simulink model "s_c_nbe_m32k"  (R2018a)
settings: Solver=VariableStepDiscrete  StartTime=0.0  StopTime=1000  RelTol=1e-3
undefined symbols (not defined in the file): fft_stages, n_taps, output_bits, pfb_coeff_gen_calc, xengbits
libraries: xbsIndex_r4 x23714, casper_library_misc x17, xps_library x4, casper_library_scopes x4, xbsReplacements_r4 x4
(part 62 of 171)

== system s_c_nbe_m32k/wb_prog_delay/delay_wideband_prog ==
  sync : Inport
  delay : Inport  Port=2
  ld_delay : Inport  Port=3
  data_in0 : Inport  Port=4
  data_in1 : Inport  Port=5
  data_in2 : Inport  Port=6
  data_in3 : Inport  Port=7
  data_in4 : Inport  Port=8
  data_in5 : Inport  Port=9
  data_in6 : Inport  Port=10
  data_in7 : Inport  Port=11
  en : Inport  Port=12
  AddSub{1..7} (7 alike) : xbsIndex_r4/AddSub  mode=Addition  use_carryin=off  use_carryout=off  en=off  latency=0  precision=Full  arith_type=Unsigned  n_bits=1  bin_pt=0  quantization=Truncate  overflow=Wrap  use_behavioral_HDL=off  hw_selection=Fabric  pipelined=off  dbl_ovrd=off  block_type=addsub
  Constant1 : xbsIndex_r4/Constant  const=6  gui_display_data_type=Fixed-point  arith_type=Unsigned  n_bits=3  bin_pt=0  preci_type=Single  exp_width=8  frac_width=24  explicit_period=on  period=1  equ=P=C  opselect=C  inp2=PCIN>>17  opr=+  inp1=P  carry=CIN  dbl_ovrd=off  block_type=constant
  Constant2 : xbsIndex_r4/Constant  const=5  gui_display_data_type=Fixed-point  arith_type=Unsigned  n_bits=3  bin_pt=0  preci_type=Single  exp_width=8  frac_width=24  explicit_period=on  period=1  equ=P=C  opselect=C  inp2=PCIN>>17  opr=+  inp1=P  carry=CIN  dbl_ovrd=off  block_type=constant
  Constant3 : xbsIndex_r4/Constant  const=4  gui_display_data_type=Fixed-point  arith_type=Unsigned  n_bits=3  bin_pt=0  preci_type=Single  exp_width=8  frac_width=24  explicit_period=on  period=1  equ=P=C  opselect=C  inp2=PCIN>>17  opr=+  inp1=P  carry=CIN  dbl_ovrd=off  block_type=constant
  Constant4 : xbsIndex_r4/Constant  const=3  gui_display_data_type=Fixed-point  arith_type=Unsigned  n_bits=3  bin_pt=0  preci_type=Single  exp_width=8  frac_width=24  explicit_period=on  period=1  equ=P=C  opselect=C  inp2=PCIN>>17  opr=+  inp1=P  carry=CIN  dbl_ovrd=off  block_type=constant
  Constant5 : xbsIndex_r4/Constant  const=2  gui_display_data_type=Fixed-point  arith_type=Unsigned  n_bits=3  bin_pt=0  preci_type=Single  exp_width=8  frac_width=24  explicit_period=on  period=1  equ=P=C  opselect=C  inp2=PCIN>>17  opr=+  inp1=P  carry=CIN  dbl_ovrd=off  block_type=constant
  Constant6 : xbsIndex_r4/Constant  const=1  gui_display_data_type=Fixed-point  arith_type=Unsigned  n_bits=3  bin_pt=0  preci_type=Single  exp_width=8  frac_width=24  explicit_period=on  period=1  equ=P=C  opselect=C  inp2=PCIN>>17  opr=+  inp1=P  carry=CIN  dbl_ovrd=off  block_type=constant
  Constant7 : xbsIndex_r4/Constant  const=0  gui_display_data_type=Fixed-point  arith_type=Unsigned  n_bits=3  bin_pt=0  preci_type=Single  exp_width=8  frac_width=24  explicit_period=on  period=1  equ=P=C  opselect=C  inp2=PCIN>>17  opr=+  inp1=P  carry=CIN  dbl_ovrd=off  block_type=constant
  Convert{1..7} (7 alike) : xbsIndex_r4/Convert  gui_display_data_type=Fixed-point  arith_type=Unsigned  n_bits=1  bin_pt=0  float_type=Single  exp_bits=8  fraction_bits=24  quantization=Truncate  overflow=Wrap  en=off  latency=0  pipeline=off  dbl_ovrd=off  block_type=convert
  Relational{1..7} (7 alike) : xbsIndex_r4/Relational  mode=a>b  op_type=Bool  en=off  latency=0  dbl_ovrd=off  block_type=relational
  barrel_switcher : Subsystem  mask(barrel_switcher){n_inputs=3, async=on}
      mask prompts: n_inputs "Number of Inputs: (2^?)"; async "Asynchronous operation"
      mask help:
      | Shifts input to right by amount specified on sel,
      | wrapping around into higher order bits.
      mask init:
      | barrel_switcher_init(gcb,...
      |     'n_inputs', n_inputs, ...
      |     'async', async);
      mask Help: eval('xlWeb(''http://casper.berkeley.edu/wiki/Barrel_switcher'')')
  bram_rd_addrs : xbsIndex_r4/Slice  nbits=1  boolean_output=off  mode=Lower Bit Location + Width  bit1=0  base1=MSB of Input  bit0=3  base0=LSB of Input  dbl_ovrd=off  block_type=slice
  delay_dp0 : Subsystem  mask(delay_bram_prog_dp){ram_bits=2, bram_latency=3, async=on}
      mask prompts: ram_bits "Max delay (2^?)"; bram_latency "BRAM latency"; async "asynchronous operation"
      mask init:
      | %delay_bram_prog_dp_init(gcb, ...
      | %    'ram_bits', ram_bits, ...
      | %    'bram_latency', bram_latency, ...
      | %    'async', async);
  delay_dp1 : Subsystem  mask(delay_bram_prog_dp){ram_bits=2, bram_latency=3, async=on}
      mask prompts: ram_bits "Max delay (2^?)"; bram_latency "BRAM latency"; async "asynchronous operation"
      mask init:
      | %delay_bram_prog_dp_init(gcb, ...
      | %    'ram_bits', ram_bits, ...
      | %    'bram_latency', bram_latency, ...
      | %    'async', async);
  delay_dp2 : Subsystem  mask(delay_bram_prog_dp){ram_bits=2, bram_latency=3, async=on}
      mask prompts: ram_bits "Max delay (2^?)"; bram_latency "BRAM latency"; async "asynchronous operation"
      mask init:
      | %delay_bram_prog_dp_init(gcb, ...
      | %    'ram_bits', ram_bits, ...
      | %    'bram_latency', bram_latency, ...
      | %    'async', async);
  delay_dp3 : Subsystem  mask(delay_bram_prog_dp){ram_bits=2, bram_latency=3, async=on}
      mask prompts: ram_bits "Max delay (2^?)"; bram_latency "BRAM latency"; async "asynchronous operation"
      mask init:
      | %delay_bram_prog_dp_init(gcb, ...
      | %    'ram_bits', ram_bits, ...
      | %    'bram_latency', bram_latency, ...
      | %    'async', async);
  delay_dp4 : Subsystem  mask(delay_bram_prog_dp){ram_bits=2, bram_latency=3, async=on}
      mask prompts: ram_bits "Max delay (2^?)"; bram_latency "BRAM latency"; async "asynchronous operation"
      mask init:
      | %delay_bram_prog_dp_init(gcb, ...
      | %    'ram_bits', ram_bits, ...
      | %    'bram_latency', bram_latency, ...
      | %    'async', async);
  delay_dp5 : Subsystem  mask(delay_bram_prog_dp){ram_bits=2, bram_latency=3, async=on}
      mask prompts: ram_bits "Max delay (2^?)"; bram_latency "BRAM latency"; async "asynchronous operation"
      mask init:
      | %delay_bram_prog_dp_init(gcb, ...
      | %    'ram_bits', ram_bits, ...
      | %    'bram_latency', bram_latency, ...
      | %    'async', async);
  delay_dp6 : Subsystem  mask(delay_bram_prog_dp){ram_bits=2, bram_latency=3, async=on}
      mask prompts: ram_bits "Max delay (2^?)"; bram_latency "BRAM latency"; async "asynchronous operation"
      mask init:
      | %delay_bram_prog_dp_init(gcb, ...
      | %    'ram_bits', ram_bits, ...
      | %    'bram_latency', bram_latency, ...
      | %    'async', async);
  delay_dp7 : Subsystem  mask(delay_bram_prog_dp){ram_bits=2, bram_latency=3, async=on}
      mask prompts: ram_bits "Max delay (2^?)"; bram_latency "BRAM latency"; async "asynchronous operation"
      mask init:
      | %delay_bram_prog_dp_init(gcb, ...
      | %    'ram_bits', ram_bits, ...
      | %    'bram_latency', bram_latency, ...
      | %    'async', async);
  delay_reg : xbsIndex_r4/Register  init=0  rst=off  en=on  dbl_ovrd=off  block_type=register
  delay_sel : xbsIndex_r4/Delay  rst=off  infoeditControl=Selection of Reset will increase slice count due to use of real FFs and instead of SRLs  en=off  latency=4  reg_retiming=on  dbl_ovrd=off  block_type=delay
  en_delay0 : xbsIndex_r4/Delay  rst=off  infoeditControl=Selection of Reset will increase slice count due to use of real FFs and instead of SRLs  en=off  latency=0  reg_retiming=on  dbl_ovrd=off  block_type=delay
  en_delay1 : xbsIndex_r4/Delay  rst=off  infoeditControl=Selection of Reset will increase slice count due to use of real FFs and instead of SRLs  en=off  latency=4  reg_retiming=on  dbl_ovrd=off  block_type=delay
  shift_sel : xbsIndex_r4/Slice  nbits=3  boolean_output=off  mode=Lower Bit Location + Width  bit1=0  base1=MSB of Input  bit0=0  base0=LSB of Input  dbl_ovrd=off  block_type=slice
  sync_delay : xbsIndex_r4/Delay  rst=off  infoeditControl=Selection of Reset will increase slice count due to use of real FFs and instead of SRLs  en=off  latency=4  reg_retiming=on  dbl_ovrd=off  block_type=delay
  sync_out : Outport
  data_out0 : Outport  Port=2
  data_out1 : Outport  Port=3
  data_out2 : Outport  Port=4
  data_out3 : Outport  Port=5
  data_out4 : Outport  Port=6
  data_out5 : Outport  Port=7
  data_out6 : Outport  Port=8
  data_out7 : Outport  Port=9
  dvalid : Outport  Port=10
  wires:
  en/1 -> en_delay0/1
  en_delay0/1 -> en_delay1/1, delay_dp0/3(en), delay_dp1/3(en), delay_dp2/3(en), delay_dp3/3(en), delay_dp4/3(en), delay_dp5/3(en), delay_dp6/3(en), delay_dp7/3(en)  "dp_en"
  sync/1 -> sync_delay/1
  delay/1 -> delay_reg/1
  ld_delay/1 -> delay_reg/2
  delay_reg/1 -> bram_rd_addrs/1, shift_sel/1
  sync_delay/1 -> barrel_switcher/2(sync_in)
  barrel_switcher/1(sync_out) -> sync_out/1
  en_delay1/1 -> barrel_switcher/11(en)
  barrel_switcher/10(dvalid) -> dvalid/1
  shift_sel/1 -> delay_sel/1, Relational1/1, Relational2/1, Relational3/1, Relational4/1, Relational5/1, Relational6/1, Relational7/1
  delay_sel/1 -> barrel_switcher/1(sel)
  barrel_switcher/9(Out8) -> data_out0/1
  barrel_switcher/8(Out7) -> data_out1/1
  barrel_switcher/7(Out6) -> data_out2/1
  barrel_switcher/6(Out5) -> data_out3/1
  barrel_switcher/5(Out4) -> data_out4/1
  barrel_switcher/4(Out3) -> data_out5/1
  barrel_switcher/3(Out2) -> data_out6/1
  barrel_switcher/2(Out1) -> data_out7/1
  data_in0/1 -> delay_dp0/1(din)  "dp_val0"
  delay_dp0/1(dout) -> barrel_switcher/10(In8)
  bram_rd_addrs/1 -> delay_dp0/2(delay), AddSub1/1, AddSub2/1, AddSub3/1, AddSub4/1, AddSub5/1, AddSub6/1, AddSub7/1  "dp0"
  data_in1/1 -> delay_dp1/1(din)  "dp_val1"
  delay_dp1/1(dout) -> barrel_switcher/9(In7)
  Constant1/1 -> Relational1/2
  Relational1/1 -> Convert1/1
  Convert1/1 -> AddSub1/2
  AddSub1/1 -> delay_dp1/2(delay)  "dp1"
  data_in2/1 -> delay_dp2/1(din)  "dp_val2"
  delay_dp2/1(dout) -> barrel_switcher/8(In6)
  Constant2/1 -> Relational2/2
  Relational2/1 -> Convert2/1
  Convert2/1 -> AddSub2/2
  AddSub2/1 -> delay_dp2/2(delay)  "dp2"
  data_in3/1 -> delay_dp3/1(din)  "dp_val3"
  delay_dp3/1(dout) -> barrel_switcher/7(In5)
  Constant3/1 -> Relational3/2
  Relational3/1 -> Convert3/1
  Convert3/1 -> AddSub3/2
  AddSub3/1 -> delay_dp3/2(delay)  "dp3"
  data_in4/1 -> delay_dp4/1(din)  "dp_val4"
  delay_dp4/1(dout) -> barrel_switcher/6(In4)
  Constant4/1 -> Relational4/2
  Relational4/1 -> Convert4/1
  Convert4/1 -> AddSub4/2
  AddSub4/1 -> delay_dp4/2(delay)  "dp4"
  data_in5/1 -> delay_dp5/1(din)  "dp_val5"
  delay_dp5/1(dout) -> barrel_switcher/5(In3)
  Constant5/1 -> Relational5/2
  Relational5/1 -> Convert5/1
  Convert5/1 -> AddSub5/2
  AddSub5/1 -> delay_dp5/2(delay)  "dp5"
  data_in6/1 -> delay_dp6/1(din)  "dp_val6"
  delay_dp6/1(dout) -> barrel_switcher/4(In2)
  Constant6/1 -> Relational6/2
  Relational6/1 -> Convert6/1
  Convert6/1 -> AddSub6/2
  AddSub6/1 -> delay_dp6/2(delay)  "dp6"
  data_in7/1 -> delay_dp7/1(din)  "dp_val7"
  delay_dp7/1(dout) -> barrel_switcher/3(In1)
  Constant7/1 -> Relational7/2
  Relational7/1 -> Convert7/1
  Convert7/1 -> AddSub7/2
  AddSub7/1 -> delay_dp7/2(delay)  "dp7"

== system s_c_nbe_m32k/wb_prog_delay1/bus_expand ==
  bus_in : Inport
  reinterpret{1..8} (8 alike) : xbsIndex_r4/Reinterpret  force_arith_type=on  arith_type=Unsigned  force_bin_pt=on  bin_pt=0  block_type=reinterpret
  slice1 : xbsIndex_r4/Slice  nbits=10  boolean_output=off  mode=Upper Bit Location + Width  bit1=-70  base1=MSB of Input  bit0=0  base0=LSB of Input  dbl_ovrd=off  block_type=slice
  slice2 : xbsIndex_r4/Slice  nbits=10  boolean_output=off  mode=Upper Bit Location + Width  bit1=-60  base1=MSB of Input  bit0=0  base0=LSB of Input  dbl_ovrd=off  block_type=slice
  slice3 : xbsIndex_r4/Slice  nbits=10  boolean_output=off  mode=Upper Bit Location + Width  bit1=-50  base1=MSB of Input  bit0=0  base0=LSB of Input  dbl_ovrd=off  block_type=slice
  slice4 : xbsIndex_r4/Slice  nbits=10  boolean_output=off  mode=Upper Bit Location + Width  bit1=-40  base1=MSB of Input  bit0=0  base0=LSB of Input  dbl_ovrd=off  block_type=slice
  slice5 : xbsIndex_r4/Slice  nbits=10  boolean_output=off  mode=Upper Bit Location + Width  bit1=-30  base1=MSB of Input  bit0=0  base0=LSB of Input  dbl_ovrd=off  block_type=slice
  slice6 : xbsIndex_r4/Slice  nbits=10  boolean_output=off  mode=Upper Bit Location + Width  bit1=-20  base1=MSB of Input  bit0=0  base0=LSB of Input  dbl_ovrd=off  block_type=slice
  slice7 : xbsIndex_r4/Slice  nbits=10  boolean_output=off  mode=Upper Bit Location + Width  bit1=-10  base1=MSB of Input  bit0=0  base0=LSB of Input  dbl_ovrd=off  block_type=slice
  slice8 : xbsIndex_r4/Slice  nbits=10  boolean_output=off  mode=Upper Bit Location + Width  bit1=0  base1=MSB of Input  bit0=0  base0=LSB of Input  dbl_ovrd=off  block_type=slice
  msb_out8 : Outport
  out7 : Outport  Port=2
  out6 : Outport  Port=3
  out5 : Outport  Port=4
  out4 : Outport  Port=5
  out3 : Outport  Port=6
  out2 : Outport  Port=7
  lsb_out1 : Outport  Port=8
  wires:
  bus_in/1 -> slice8/1, slice7/1, slice6/1, slice5/1, slice4/1, slice3/1, slice2/1, slice1/1
  slice8/1 -> reinterpret8/1
  reinterpret8/1 -> msb_out8/1
  slice7/1 -> reinterpret7/1
  reinterpret7/1 -> out7/1
  slice6/1 -> reinterpret6/1
  reinterpret6/1 -> out6/1
  slice5/1 -> reinterpret5/1
  reinterpret5/1 -> out5/1
  slice4/1 -> reinterpret4/1
  reinterpret4/1 -> out4/1
  slice3/1 -> reinterpret3/1
  reinterpret3/1 -> out3/1
  slice2/1 -> reinterpret2/1
  reinterpret2/1 -> out2/1
  slice1/1 -> reinterpret1/1
  reinterpret1/1 -> lsb_out1/1

== system s_c_nbe_m32k/wb_prog_delay1/bus_expand1 ==
  bus_in : Inport
  reinterpret1 : xbsIndex_r4/Reinterpret  force_arith_type=on  arith_type="Signed  (2's comp)"  force_bin_pt=on  bin_pt=15  block_type=reinterpret
  reinterpret2 : xbsIndex_r4/Reinterpret  force_arith_type=on  arith_type="Signed  (2's comp)"  force_bin_pt=on  bin_pt=15  block_type=reinterpret
  reinterpret3 : xbsIndex_r4/Reinterpret  force_arith_type=on  arith_type="Signed  (2's comp)"  force_bin_pt=on  bin_pt=32  block_type=reinterpret
  reinterpret4 : xbsIndex_r4/Reinterpret  force_arith_type=on  arith_type="Signed  (2's comp)"  force_bin_pt=on  bin_pt=32  block_type=reinterpret
  slice1 : xbsIndex_r4/Slice  nbits=16  boolean_output=off  mode=Upper Bit Location + Width  bit1=-144  base1=MSB of Input  bit0=0  base0=LSB of Input  dbl_ovrd=off  block_type=slice
  slice2 : xbsIndex_r4/Slice  nbits=16  boolean_output=off  mode=Upper Bit Location + Width  bit1=-128  base1=MSB of Input  bit0=0  base0=LSB of Input  dbl_ovrd=off  block_type=slice
  slice3 : xbsIndex_r4/Slice  nbits=64  boolean_output=off  mode=Upper Bit Location + Width  bit1=-64  base1=MSB of Input  bit0=0  base0=LSB of Input  dbl_ovrd=off  block_type=slice
  slice4 : xbsIndex_r4/Slice  nbits=64  boolean_output=off  mode=Upper Bit Location + Width  bit1=0  base1=MSB of Input  bit0=0  base0=LSB of Input  dbl_ovrd=off  block_type=slice
  msb_out4 : Outport
  out3 : Outport  Port=2
  out2 : Outport  Port=3
  lsb_out1 : Outport  Port=4
  wires:
  reinterpret1/1 -> lsb_out1/1
  slice1/1 -> reinterpret1/1
  reinterpret2/1 -> out2/1
  slice2/1 -> reinterpret2/1
  reinterpret3/1 -> out3/1
  slice3/1 -> reinterpret3/1
  reinterpret4/1 -> msb_out4/1
  slice4/1 -> reinterpret4/1
  bus_in/1 -> slice1/1, slice2/1, slice3/1, slice4/1

== system s_c_nbe_m32k/wb_prog_delay1/delay_gen ==
  sync_in : Inport
  din : Inport  Port=2
  en : Inport  Port=3
  delay : Inport  Port=4
  d/dt_delay : Inport  Port=5
  phase : Inport  Port=6
  d/dt_phase : Inport  Port=7
  ld : Inport  Port=8
  Constant : xbsIndex_r4/Constant  const=2^(n_bits_fft_words-1)  gui_display_data_type=Fixed-point  arith_type=Unsigned  n_bits=n_bits_fft_words  bin_pt=0  preci_type=Single  exp_width=8  frac_width=24  explicit_period=on  period=1  equ=P=C  opselect=C  inp2=PCIN>>17  opr=+  inp1=P  carry=CIN  dbl_ovrd=off  block_type=constant
  Constant53 : xbsIndex_r4/Constant  const=0  gui_display_data_type=Boolean  arith_type=Boolean  n_bits=1  bin_pt=0  preci_type=Single  exp_width=8  frac_width=24  explicit_period=on  period=1  equ=P=C  opselect=C  inp2=PCIN>>17  opr=+  inp1=P  carry=CIN  dbl_ovrd=off  block_type=constant
      settings: block_version=11.4
  Delay{,1..17} (18 alike) : xbsIndex_r4/Delay  rst=off  infoeditControl=Selection of Reset will increase slice count due to use of real FFs and instead of SRLs  en=off  latency=1  reg_retiming=on  dbl_ovrd=off  block_type=delay
  Logical : xbsIndex_r4/Logical  logical_function=AND  inputs=2  en=off  latency=1  precision=Full  arith_type=Unsigned  n_bits=16  bin_pt=0  align_bp=on  dbl_ovrd=off  block_type=logical
  delay_gen : Subsystem  mask{fft_len=n_bits_fft, add_latency=1, data_bits=n_bits_data * 2^n_bits_streams, n_bits_index=n_bits_fft_words, lookup_bits=11, cd_bits=n_bits_cd, delay_bits=n_bits_cd+32, delay_bin_pt=32, max_delay_rate=23, min_delay_rate=38, phase_bits=16, max_phase_rate=23, min_phase_rate=38}
      mask prompts: fft_len "Effective FFT size (2^?)"; add_latency "Add latency"; data_bits "Data width"; n_bits_index "Index width"; lookup_bits "DDS lookup table resolution (2*pi/2^?)"; cd_bits "Coarse delay range (2^? bits)"; delay_bits "Input delay resolution (bits)"; delay_bin_pt "Input delay binary point"; max_delay_rate "Max delay update rate (1/2^? samples/sample)"; min_delay_rate "Min (non-zero) delay update rate (1/2^? samples/sample)"; phase_bits "Input phase resolution (2*pi/2^? radians)"; max_phase_rate "Max phase update rate (1/2^? radians/sample)"; min_phase_rate "Min (non-zero) phase rate (1/2^? radians/sample)"
  edge_detect : Subsystem  mask(edge_detect){edge=Rising, polarity=Active High, x_in=[0 0.08 0.08 0.16 0.16 0.24 0.24 0.32 0.32 0.4], y_in=[-1 -1  1  1  1  1  1  1  1  1], x_out=[0.6 0.68 0.68 0.76 0.76 0.84 0.84 0.92 0.92 1], y_out=[-1 -1  1  1 -1 -1 -1 -1 -1 -1]}
      mask prompts: edge "Edge Type"; polarity "Output Polarity"; x_in "Input X Positions"; y_in "Input Y Positions"; x_out "Output X Positions"; y_out "Output Y Positions"
      mask help: Output is active for one-cycle after each edge of the specified type (i.e. rising, falling or both).
      mask init: same as s_c_nbe_m32k/edge_detect1
      settings: AttributesFormatString=|
      | rising edges
      | active high
      mask Help: Output is active for one-cycle after each edge of the specified type (i.e. rising, falling, or both).  Latency is zero.
      mask TypeOptions edge: Rising | Falling | Both
      mask TypeOptions polarity: Active High | Active Low
      mask Display:
      | plot(x_in_num,0.5+y_in_num*0.2);
      | plot(x_out_num,0.5+y_out_num*0.2);
  fft_index : xbsIndex_r4/Counter  cnt_type=Free Running  cnt_to=Inf  operation=Up  start_count=2^(n_bits_fft_words-1)  cnt_by_val=1  arith_type=Unsigned  n_bits=n_bits_fft_words  bin_pt=0  load_pin=off  rst=on  en=on  explicit_period=on  period=1  use_behavioral_HDL=on  implementation=Fabric  dbl_ovrd=off  block_type=counter
  first : xbsIndex_r4/Relational  mode=a=b  op_type=Bool  en=off  latency=1  dbl_ovrd=off  block_type=relational
  sync_out : Outport
  dout : Outport  Port=2
  idx_out : Outport  Port=3
  dvalid : Outport  Port=4
  initial_phase : Outport  Port=5
  slope : Outport  Port=6
  coarse_delay : Outport  Port=7
  new_value : Outport  Port=8
  wires:
  edge_detect/1(out) -> delay_gen/2(init)
  Logical/1 -> edge_detect/1(in)
  Delay17/1 -> delay_gen/10(d/dt_delay)
  Delay16/1 -> delay_gen/9(delay)
  Delay15/1 -> delay_gen/8(d/dt_phase)
  Delay14/1 -> delay_gen/7(phase)
  Delay13/1 -> delay_gen/6(load)
  Delay12/1 -> delay_gen/5(den)
  Delay11/1 -> delay_gen/4(idx_in)
  Delay10/1 -> delay_gen/3(din)
  Delay9/1 -> delay_gen/1(sync_in)
  Delay1/1 -> Delay10/1
  Delay8/1 -> Delay17/1
  Delay7/1 -> Delay16/1
  Delay6/1 -> Delay15/1
  Delay5/1 -> Delay14/1
  Delay4/1 -> Delay13/1
  delay_gen/8(load_out) -> new_value/1
  delay_gen/7(phase_out) -> initial_phase/1
  delay_gen/6(slope_out) -> slope/1
  delay_gen/5(cd_o) -> coarse_delay/1
  delay_gen/4(dvalid) -> dvalid/1
  delay_gen/3(idx_out) -> idx_out/1
  d/dt_phase/1 -> Delay6/1
  phase/1 -> Delay5/1
  ld/1 -> Delay4/1
  Delay3/1 -> Delay12/1, Logical/2
  Delay2/1 -> Delay11/1
  Delay/1 -> Delay9/1
  first/1 -> Logical/1
  Constant/1 -> first/1
  delay_gen/2(dout) -> dout/1
  en/1 -> fft_index/2, Delay3/1
  d/dt_delay/1 -> Delay8/1
  delay_gen/1(sync_out) -> sync_out/1
  delay/1 -> Delay7/1
  fft_index/1 -> first/2, Delay2/1
  Constant53/1 -> delay_gen/11(invert_slope)
  sync_in/1 -> fft_index/1, Delay/1
  din/1 -> Delay1/1

== system s_c_nbe_m32k/wb_prog_delay1/delay_wideband_prog ==
  sync : Inport
  delay : Inport  Port=2
  ld_delay : Inport  Port=3
  data_in0 : Inport  Port=4
  data_in1 : Inport  Port=5
  data_in2 : Inport  Port=6
  data_in3 : Inport  Port=7
  data_in4 : Inport  Port=8
  data_in5 : Inport  Port=9
  data_in6 : Inport  Port=10
  data_in7 : Inport  Port=11
  en : Inport  Port=12
  AddSub{1..7} (7 alike) : xbsIndex_r4/AddSub  mode=Addition  use_carryin=off  use_carryout=off  en=off  latency=0  precision=Full  arith_type=Unsigned  n_bits=1  bin_pt=0  quantization=Truncate  overflow=Wrap  use_behavioral_HDL=off  hw_selection=Fabric  pipelined=off  dbl_ovrd=off  block_type=addsub
  Constant1 : xbsIndex_r4/Constant  const=6  gui_display_data_type=Fixed-point  arith_type=Unsigned  n_bits=3  bin_pt=0  preci_type=Single  exp_width=8  frac_width=24  explicit_period=on  period=1  equ=P=C  opselect=C  inp2=PCIN>>17  opr=+  inp1=P  carry=CIN  dbl_ovrd=off  block_type=constant
  Constant2 : xbsIndex_r4/Constant  const=5  gui_display_data_type=Fixed-point  arith_type=Unsigned  n_bits=3  bin_pt=0  preci_type=Single  exp_width=8  frac_width=24  explicit_period=on  period=1  equ=P=C  opselect=C  inp2=PCIN>>17  opr=+  inp1=P  carry=CIN  dbl_ovrd=off  block_type=constant
  Constant3 : xbsIndex_r4/Constant  const=4  gui_display_data_type=Fixed-point  arith_type=Unsigned  n_bits=3  bin_pt=0  preci_type=Single  exp_width=8  frac_width=24  explicit_period=on  period=1  equ=P=C  opselect=C  inp2=PCIN>>17  opr=+  inp1=P  carry=CIN  dbl_ovrd=off  block_type=constant
  Constant4 : xbsIndex_r4/Constant  const=3  gui_display_data_type=Fixed-point  arith_type=Unsigned  n_bits=3  bin_pt=0  preci_type=Single  exp_width=8  frac_width=24  explicit_period=on  period=1  equ=P=C  opselect=C  inp2=PCIN>>17  opr=+  inp1=P  carry=CIN  dbl_ovrd=off  block_type=constant
  Constant5 : xbsIndex_r4/Constant  const=2  gui_display_data_type=Fixed-point  arith_type=Unsigned  n_bits=3  bin_pt=0  preci_type=Single  exp_width=8  frac_width=24  explicit_period=on  period=1  equ=P=C  opselect=C  inp2=PCIN>>17  opr=+  inp1=P  carry=CIN  dbl_ovrd=off  block_type=constant
  Constant6 : xbsIndex_r4/Constant  const=1  gui_display_data_type=Fixed-point  arith_type=Unsigned  n_bits=3  bin_pt=0  preci_type=Single  exp_width=8  frac_width=24  explicit_period=on  period=1  equ=P=C  opselect=C  inp2=PCIN>>17  opr=+  inp1=P  carry=CIN  dbl_ovrd=off  block_type=constant
  Constant7 : xbsIndex_r4/Constant  const=0  gui_display_data_type=Fixed-point  arith_type=Unsigned  n_bits=3  bin_pt=0  preci_type=Single  exp_width=8  frac_width=24  explicit_period=on  period=1  equ=P=C  opselect=C  inp2=PCIN>>17  opr=+  inp1=P  carry=CIN  dbl_ovrd=off  block_type=constant
  Convert{1..7} (7 alike) : xbsIndex_r4/Convert  gui_display_data_type=Fixed-point  arith_type=Unsigned  n_bits=1  bin_pt=0  float_type=Single  exp_bits=8  fraction_bits=24  quantization=Truncate  overflow=Wrap  en=off  latency=0  pipeline=off  dbl_ovrd=off  block_type=convert
  Relational{1..7} (7 alike) : xbsIndex_r4/Relational  mode=a>b  op_type=Bool  en=off  latency=0  dbl_ovrd=off  block_type=relational
  barrel_switcher : Subsystem  mask(barrel_switcher){n_inputs=3, async=on}
      mask prompts: n_inputs "Number of Inputs: (2^?)"; async "Asynchronous operation"
      mask help:
      | Shifts input to right by amount specified on sel,
      | wrapping around into higher order bits.
      mask init:
      | barrel_switcher_init(gcb,...
      |     'n_inputs', n_inputs, ...
      |     'async', async);
      mask Help: eval('xlWeb(''http://casper.berkeley.edu/wiki/Barrel_switcher'')')
  bram_rd_addrs : xbsIndex_r4/Slice  nbits=1  boolean_output=off  mode=Lower Bit Location + Width  bit1=0  base1=MSB of Input  bit0=3  base0=LSB of Input  dbl_ovrd=off  block_type=slice
  delay_dp0 : Subsystem  mask(delay_bram_prog_dp){ram_bits=2, bram_latency=3, async=on}
      mask prompts: ram_bits "Max delay (2^?)"; bram_latency "BRAM latency"; async "asynchronous operation"
      mask init:
      | %delay_bram_prog_dp_init(gcb, ...
      | %    'ram_bits', ram_bits, ...
      | %    'bram_latency', bram_latency, ...
      | %    'async', async);
  delay_dp1 : Subsystem  mask(delay_bram_prog_dp){ram_bits=2, bram_latency=3, async=on}
      mask prompts: ram_bits "Max delay (2^?)"; bram_latency "BRAM latency"; async "asynchronous operation"
      mask init:
      | %delay_bram_prog_dp_init(gcb, ...
      | %    'ram_bits', ram_bits, ...
      | %    'bram_latency', bram_latency, ...
      | %    'async', async);
  delay_dp2 : Subsystem  mask(delay_bram_prog_dp){ram_bits=2, bram_latency=3, async=on}
      mask prompts: ram_bits "Max delay (2^?)"; bram_latency "BRAM latency"; async "asynchronous operation"
      mask init:
      | %delay_bram_prog_dp_init(gcb, ...
      | %    'ram_bits', ram_bits, ...
      | %    'bram_latency', bram_latency, ...
      | %    'async', async);
  delay_dp3 : Subsystem  mask(delay_bram_prog_dp){ram_bits=2, bram_latency=3, async=on}
      mask prompts: ram_bits "Max delay (2^?)"; bram_latency "BRAM latency"; async "asynchronous operation"
      mask init:
      | %delay_bram_prog_dp_init(gcb, ...
      | %    'ram_bits', ram_bits, ...
      | %    'bram_latency', bram_latency, ...
      | %    'async', async);
  delay_dp4 : Subsystem  mask(delay_bram_prog_dp){ram_bits=2, bram_latency=3, async=on}
      mask prompts: ram_bits "Max delay (2^?)"; bram_latency "BRAM latency"; async "asynchronous operation"
      mask init:
      | %delay_bram_prog_dp_init(gcb, ...
      | %    'ram_bits', ram_bits, ...
      | %    'bram_latency', bram_latency, ...
      | %    'async', async);
  delay_dp5 : Subsystem  mask(delay_bram_prog_dp){ram_bits=2, bram_latency=3, async=on}
      mask prompts: ram_bits "Max delay (2^?)"; bram_latency "BRAM latency"; async "asynchronous operation"
      mask init:
      | %delay_bram_prog_dp_init(gcb, ...
      | %    'ram_bits', ram_bits, ...
      | %    'bram_latency', bram_latency, ...
      | %    'async', async);
  delay_dp6 : Subsystem  mask(delay_bram_prog_dp){ram_bits=2, bram_latency=3, async=on}
      mask prompts: ram_bits "Max delay (2^?)"; bram_latency "BRAM latency"; async "asynchronous operation"
      mask init:
      | %delay_bram_prog_dp_init(gcb, ...
      | %    'ram_bits', ram_bits, ...
      | %    'bram_latency', bram_latency, ...
      | %    'async', async);
  delay_dp7 : Subsystem  mask(delay_bram_prog_dp){ram_bits=2, bram_latency=3, async=on}
      mask prompts: ram_bits "Max delay (2^?)"; bram_latency "BRAM latency"; async "asynchronous operation"
      mask init:
      | %delay_bram_prog_dp_init(gcb, ...
      | %    'ram_bits', ram_bits, ...
      | %    'bram_latency', bram_latency, ...
      | %    'async', async);
  delay_reg : xbsIndex_r4/Register  init=0  rst=off  en=on  dbl_ovrd=off  block_type=register
  delay_sel : xbsIndex_r4/Delay  rst=off  infoeditControl=Selection of Reset will increase slice count due to use of real FFs and instead of SRLs  en=off  latency=4  reg_retiming=on  dbl_ovrd=off  block_type=delay
  en_delay0 : xbsIndex_r4/Delay  rst=off  infoeditControl=Selection of Reset will increase slice count due to use of real FFs and instead of SRLs  en=off  latency=0  reg_retiming=on  dbl_ovrd=off  block_type=delay
  en_delay1 : xbsIndex_r4/Delay  rst=off  infoeditControl=Selection of Reset will increase slice count due to use of real FFs and instead of SRLs  en=off  latency=4  reg_retiming=on  dbl_ovrd=off  block_type=delay
  shift_sel : xbsIndex_r4/Slice  nbits=3  boolean_output=off  mode=Lower Bit Location + Width  bit1=0  base1=MSB of Input  bit0=0  base0=LSB of Input  dbl_ovrd=off  block_type=slice
  sync_delay : xbsIndex_r4/Delay  rst=off  infoeditControl=Selection of Reset will increase slice count due to use of real FFs and instead of SRLs  en=off  latency=4  reg_retiming=on  dbl_ovrd=off  block_type=delay
  sync_out : Outport
  data_out0 : Outport  Port=2
  data_out1 : Outport  Port=3
  data_out2 : Outport  Port=4
  data_out3 : Outport  Port=5
  data_out4 : Outport  Port=6
  data_out5 : Outport  Port=7
  data_out6 : Outport  Port=8
  data_out7 : Outport  Port=9
  dvalid : Outport  Port=10
  wires:
  AddSub7/1 -> delay_dp7/2(delay)  "dp7"
  Convert7/1 -> AddSub7/2
  Relational7/1 -> Convert7/1
  Constant7/1 -> Relational7/2
  delay_dp7/1(dout) -> barrel_switcher/3(In1)
  data_in7/1 -> delay_dp7/1(din)  "dp_val7"
  AddSub6/1 -> delay_dp6/2(delay)  "dp6"
  Convert6/1 -> AddSub6/2
  Relational6/1 -> Convert6/1
  Constant6/1 -> Relational6/2
  delay_dp6/1(dout) -> barrel_switcher/4(In2)
  data_in6/1 -> delay_dp6/1(din)  "dp_val6"
  AddSub5/1 -> delay_dp5/2(delay)  "dp5"
  Convert5/1 -> AddSub5/2
  Relational5/1 -> Convert5/1
  Constant5/1 -> Relational5/2
  delay_dp5/1(dout) -> barrel_switcher/5(In3)
  data_in5/1 -> delay_dp5/1(din)  "dp_val5"
  AddSub4/1 -> delay_dp4/2(delay)  "dp4"
  Convert4/1 -> AddSub4/2
  Relational4/1 -> Convert4/1
  Constant4/1 -> Relational4/2
  delay_dp4/1(dout) -> barrel_switcher/6(In4)
  data_in4/1 -> delay_dp4/1(din)  "dp_val4"
  AddSub3/1 -> delay_dp3/2(delay)  "dp3"
  Convert3/1 -> AddSub3/2
  Relational3/1 -> Convert3/1
  Constant3/1 -> Relational3/2
  delay_dp3/1(dout) -> barrel_switcher/7(In5)
  data_in3/1 -> delay_dp3/1(din)  "dp_val3"
  AddSub2/1 -> delay_dp2/2(delay)  "dp2"
  Convert2/1 -> AddSub2/2
  Relational2/1 -> Convert2/1
  Constant2/1 -> Relational2/2
  delay_dp2/1(dout) -> barrel_switcher/8(In6)
  data_in2/1 -> delay_dp2/1(din)  "dp_val2"
  AddSub1/1 -> delay_dp1/2(delay)  "dp1"
  Convert1/1 -> AddSub1/2
  Relational1/1 -> Convert1/1
  Constant1/1 -> Relational1/2
  delay_dp1/1(dout) -> barrel_switcher/9(In7)
  data_in1/1 -> delay_dp1/1(din)  "dp_val1"
  bram_rd_addrs/1 -> AddSub7/1, AddSub6/1, AddSub5/1, AddSub4/1, AddSub3/1, AddSub2/1, AddSub1/1, delay_dp0/2(delay)  "dp0"
  delay_dp0/1(dout) -> barrel_switcher/10(In8)
  data_in0/1 -> delay_dp0/1(din)  "dp_val0"
  barrel_switcher/2(Out1) -> data_out7/1
  barrel_switcher/3(Out2) -> data_out6/1
  barrel_switcher/4(Out3) -> data_out5/1
  barrel_switcher/5(Out4) -> data_out4/1
  barrel_switcher/6(Out5) -> data_out3/1
  barrel_switcher/7(Out6) -> data_out2/1
  barrel_switcher/8(Out7) -> data_out1/1
  barrel_switcher/9(Out8) -> data_out0/1
  delay_sel/1 -> barrel_switcher/1(sel)
  shift_sel/1 -> Relational7/1, Relational6/1, Relational5/1, Relational4/1, Relational3/1, Relational2/1, Relational1/1, delay_sel/1
  barrel_switcher/10(dvalid) -> dvalid/1
  en_delay1/1 -> barrel_switcher/11(en)
  barrel_switcher/1(sync_out) -> sync_out/1
  sync_delay/1 -> barrel_switcher/2(sync_in)
  delay_reg/1 -> shift_sel/1, bram_rd_addrs/1
  ld_delay/1 -> delay_reg/2
  delay/1 -> delay_reg/1
  sync/1 -> sync_delay/1
  en_delay0/1 -> delay_dp7/3(en), delay_dp6/3(en), delay_dp5/3(en), delay_dp4/3(en), delay_dp3/3(en), delay_dp2/3(en), delay_dp1/3(en), delay_dp0/3(en), en_delay1/1  "dp_en"
  en/1 -> en_delay0/1

== system s_c_nbe_m32k/DDC/bus_mult/a*b_bussify ==
  in1 : Inport
  in2 : Inport  Port=2
  in3 : Inport  Port=3
  in4 : Inport  Port=4
  in5 : Inport  Port=5
  in6 : Inport  Port=6
  in7 : Inport  Port=7
  in8 : Inport  Port=8
  concatenate : xbsIndex_r4/Concat  num_inputs=8  dbl_ovrd=off  block_type=concat
  reinterpret{1..8} (8 alike) : xbsIndex_r4/Reinterpret  force_arith_type=on  arith_type=Unsigned  force_bin_pt=on  bin_pt=0  block_type=reinterpret
      reinterpret1 settings: infoedit="Changes signal type without altering the binary representation.   You can changed the signal between signed and unsigned, and relocate the binary point.<br><br>Hardware notes: In hardware this block costs nothing.<br><br>Example:  Suppose the input is 6 bits wide, signed, with 2 fractional bits, and the output is forced to unsigned with 0 fractional bits.  Then an input of -2.0 (1110.00 in binary 2's complement) becomes an output of 56 (111000 in binary)."
      reinterpret2 settings: infoedit="Changes signal type without altering the binary representation.   You can changed the signal between signed and unsigned, and relocate the binary point.<br><br>Hardware notes: In hardware this block costs nothing.<br><br>Example:  Suppose the input is 6 bits wide, signed, with 2 fractional bits, and the output is forced to unsigned with 0 fractional bits.  Then an input of -2.0 (1110.00 in binary 2's complement) becomes an output of 56 (111000 in binary)."
  bus_out : Outport
  wires:
  concatenate/1 -> bus_out/1
  in1/1 -> reinterpret1/1
  reinterpret1/1 -> concatenate/1
  in2/1 -> reinterpret2/1
  reinterpret2/1 -> concatenate/2
  in3/1 -> reinterpret3/1
  reinterpret3/1 -> concatenate/3
  in4/1 -> reinterpret4/1
  reinterpret4/1 -> concatenate/4
  in5/1 -> reinterpret5/1
  reinterpret5/1 -> concatenate/5
  in6/1 -> reinterpret6/1
  reinterpret6/1 -> concatenate/6
  in7/1 -> reinterpret7/1
  reinterpret7/1 -> concatenate/7
  in8/1 -> reinterpret8/1
  reinterpret8/1 -> concatenate/8

== system s_c_nbe_m32k/DDC/bus_mult/a_debus ==
  bus_in : Inport
  reinterpret{1..8} (8 alike) : xbsIndex_r4/Reinterpret  force_arith_type=on  arith_type=Unsigned  force_bin_pt=on  bin_pt=0  block_type=reinterpret
  slice1 : xbsIndex_r4/Slice  nbits=20  boolean_output=off  mode=Upper Bit Location + Width  bit1=-140  base1=MSB of Input  bit0=0  base0=LSB of Input  dbl_ovrd=off  block_type=slice
  slice2 : xbsIndex_r4/Slice  nbits=20  boolean_output=off  mode=Upper Bit Location + Width  bit1=-120  base1=MSB of Input  bit0=0  base0=LSB of Input  dbl_ovrd=off  block_type=slice
  slice3 : xbsIndex_r4/Slice  nbits=20  boolean_output=off  mode=Upper Bit Location + Width  bit1=-100  base1=MSB of Input  bit0=0  base0=LSB of Input  dbl_ovrd=off  block_type=slice
  slice4 : xbsIndex_r4/Slice  nbits=20  boolean_output=off  mode=Upper Bit Location + Width  bit1=-80  base1=MSB of Input  bit0=0  base0=LSB of Input  dbl_ovrd=off  block_type=slice
  slice5 : xbsIndex_r4/Slice  nbits=20  boolean_output=off  mode=Upper Bit Location + Width  bit1=-60  base1=MSB of Input  bit0=0  base0=LSB of Input  dbl_ovrd=off  block_type=slice
  slice6 : xbsIndex_r4/Slice  nbits=20  boolean_output=off  mode=Upper Bit Location + Width  bit1=-40  base1=MSB of Input  bit0=0  base0=LSB of Input  dbl_ovrd=off  block_type=slice
  slice7 : xbsIndex_r4/Slice  nbits=20  boolean_output=off  mode=Upper Bit Location + Width  bit1=-20  base1=MSB of Input  bit0=0  base0=LSB of Input  dbl_ovrd=off  block_type=slice
  slice8 : xbsIndex_r4/Slice  nbits=20  boolean_output=off  mode=Upper Bit Location + Width  bit1=0  base1=MSB of Input  bit0=0  base0=LSB of Input  dbl_ovrd=off  block_type=slice
  msb_out8 : Outport
  out7 : Outport  Port=2
  out6 : Outport  Port=3
  out5 : Outport  Port=4
  out4 : Outport  Port=5
  out3 : Outport  Port=6
  out2 : Outport  Port=7
  lsb_out1 : Outport  Port=8
  wires:
  bus_in/1 -> slice8/1, slice7/1, slice6/1, slice5/1, slice4/1, slice3/1, slice2/1, slice1/1
  slice8/1 -> reinterpret8/1
  reinterpret8/1 -> msb_out8/1
  slice7/1 -> reinterpret7/1
  reinterpret7/1 -> out7/1
  slice6/1 -> reinterpret6/1
  reinterpret6/1 -> out6/1
  slice5/1 -> reinterpret5/1
  reinterpret5/1 -> out5/1
  slice4/1 -> reinterpret4/1
  reinterpret4/1 -> out4/1
  slice3/1 -> reinterpret3/1
  reinterpret3/1 -> out3/1
  slice2/1 -> reinterpret2/1
  reinterpret2/1 -> out2/1
  slice1/1 -> reinterpret1/1
  reinterpret1/1 -> lsb_out1/1

== system s_c_nbe_m32k/DDC/bus_mult/b_debus ==
  bus_in : Inport
  reinterpret{1..8} (8 alike) : xbsIndex_r4/Reinterpret  force_arith_type=on  arith_type=Unsigned  force_bin_pt=on  bin_pt=0  block_type=reinterpret
  slice1 : xbsIndex_r4/Slice  nbits=36  boolean_output=off  mode=Upper Bit Location + Width  bit1=-252  base1=MSB of Input  bit0=0  base0=LSB of Input  dbl_ovrd=off  block_type=slice
  slice2 : xbsIndex_r4/Slice  nbits=36  boolean_output=off  mode=Upper Bit Location + Width  bit1=-216  base1=MSB of Input  bit0=0  base0=LSB of Input  dbl_ovrd=off  block_type=slice
  slice3 : xbsIndex_r4/Slice  nbits=36  boolean_output=off  mode=Upper Bit Location + Width  bit1=-180  base1=MSB of Input  bit0=0  base0=LSB of Input  dbl_ovrd=off  block_type=slice
  slice4 : xbsIndex_r4/Slice  nbits=36  boolean_output=off  mode=Upper Bit Location + Width  bit1=-144  base1=MSB of Input  bit0=0  base0=LSB of Input  dbl_ovrd=off  block_type=slice
  slice5 : xbsIndex_r4/Slice  nbits=36  boolean_output=off  mode=Upper Bit Location + Width  bit1=-108  base1=MSB of Input  bit0=0  base0=LSB of Input  dbl_ovrd=off  block_type=slice
  slice6 : xbsIndex_r4/Slice  nbits=36  boolean_output=off  mode=Upper Bit Location + Width  bit1=-72  base1=MSB of Input  bit0=0  base0=LSB of Input  dbl_ovrd=off  block_type=slice
  slice7 : xbsIndex_r4/Slice  nbits=36  boolean_output=off  mode=Upper Bit Location + Width  bit1=-36  base1=MSB of Input  bit0=0  base0=LSB of Input  dbl_ovrd=off  block_type=slice
  slice8 : xbsIndex_r4/Slice  nbits=36  boolean_output=off  mode=Upper Bit Location + Width  bit1=0  base1=MSB of Input  bit0=0  base0=LSB of Input  dbl_ovrd=off  block_type=slice
  msb_out8 : Outport
  out7 : Outport  Port=2
  out6 : Outport  Port=3
  out5 : Outport  Port=4
  out4 : Outport  Port=5
  out3 : Outport  Port=6
  out2 : Outport  Port=7
  lsb_out1 : Outport  Port=8
  wires:
  bus_in/1 -> slice8/1, slice7/1, slice6/1, slice5/1, slice4/1, slice3/1, slice2/1, slice1/1
  slice8/1 -> reinterpret8/1
  reinterpret8/1 -> msb_out8/1
  slice7/1 -> reinterpret7/1
  reinterpret7/1 -> out7/1
  slice6/1 -> reinterpret6/1
  reinterpret6/1 -> out6/1
  slice5/1 -> reinterpret5/1
  reinterpret5/1 -> out5/1
  slice4/1 -> reinterpret4/1
  reinterpret4/1 -> out4/1
  slice3/1 -> reinterpret3/1
  reinterpret3/1 -> out3/1
  slice2/1 -> reinterpret2/1
  reinterpret2/1 -> out2/1
  slice1/1 -> reinterpret1/1
  reinterpret1/1 -> lsb_out1/1

== system s_c_nbe_m32k/DDC/bus_mult/mult1 ==
  a : Inport
  b : Inport  Port=2
  a_expand : Subsystem  mask(bus_expand){mode=divisions of equal size, outputNum=4, outputWidth=[10 10 10 10], outputBinaryPt=[9 9 9 9], outputArithmeticType=[1 1 1 1], show_format=off, outputToWorkspace=off, variablePrefix=out, outputToModelAsWell=on}
      mask prompts: outputNum "Number of outputs:"; outputWidth "Output width:"; outputBinaryPt "Output binary point position:"; outputArithmeticType "Output arithmetic type (ufix=0, fix=1, bool=2):"; show_format "Print format string?"; outputToWorkspace "Output to workspace?"; variablePrefix "Variable name prefix:"; outputToModelAsWell "Output to model as well?"
      mask help:
      | Expands a 'bus' made using a bus_create or Xilinx
      | concat block.
      | The input will be divided into the specified number
      | of outputs with the specified arithmetic types.
      | Divisions are made from most significant bit.
      mask init: same as s_c_nbe_m32k/bus_expand1
      settings: AttributesFormatString=4 outputs
      mask TypeOptions mode: divisions of equal size | divisions of arbitrary size
      mask Callback mode: bus_expand_callback();
      mask Callback outputWidth: bus_expand_callback();
      mask Callback outputToWorkspace: bus_expand_callback();
  a_replicate : Subsystem  mask(bus_replicate){replication=2, csp_latency=1, misc=off, implementation=core}
      mask prompts: replication "replication factor"; csp_latency "latency"; misc "misc support"; implementation "delay implementation"
      mask help: Output bus formed by replicating input bus a number of times
      mask init:
      | bus_replicate_init(gcb, ...
      |     'replication', replication, ...
      |     'csp_latency', csp_latency, ...
      |     'implementation', implementation, ...
      |     'misc', misc);
      mask TypeOptions implementation: core | behavioral
  addsub_im : xbsIndex_r4/AddSub  mode=Addition  use_carryin=off  use_carryout=off  en=off  latency=7  precision=Full  arith_type=Unsigned  n_bits=16  bin_pt=14  quantization=Truncate  overflow=Wrap  use_behavioral_HDL=on  hw_selection=Fabric  pipelined=on  use_rpm=on  dbl_ovrd=off  block_type=addsub
  addsub_re : xbsIndex_r4/AddSub  mode=Subtraction  use_carryin=off  use_carryout=off  en=off  latency=7  precision=Full  arith_type=Unsigned  n_bits=16  bin_pt=14  quantization=Truncate  overflow=Wrap  use_behavioral_HDL=on  hw_selection=Fabric  pipelined=on  use_rpm=on  dbl_ovrd=off  block_type=addsub
  b_expand : Subsystem  mask(bus_expand){mode=divisions of equal size, outputNum=4, outputWidth=[18 18 18 18], outputBinaryPt=[17 17 17 17], outputArithmeticType=[1 1 1 1], show_format=off, outputToWorkspace=off, variablePrefix=out, outputToModelAsWell=on}
      mask prompts: outputNum "Number of outputs:"; outputWidth "Output width:"; outputBinaryPt "Output binary point position:"; outputArithmeticType "Output arithmetic type (ufix=0, fix=1, bool=2):"; show_format "Print format string?"; outputToWorkspace "Output to workspace?"; variablePrefix "Variable name prefix:"; outputToModelAsWell "Output to model as well?"
      mask help:
      | Expands a 'bus' made using a bus_create or Xilinx
      | concat block.
      | The input will be divided into the specified number
      | of outputs with the specified arithmetic types.
      | Divisions are made from most significant bit.
      mask init: same as s_c_nbe_m32k/bus_expand1
      settings: AttributesFormatString=4 outputs
      mask TypeOptions mode: divisions of equal size | divisions of arbitrary size
      mask Callback mode: bus_expand_callback();
      mask Callback outputWidth: bus_expand_callback();
      mask Callback outputToWorkspace: bus_expand_callback();
  b_replicate : Subsystem  mask(bus_replicate){replication=2, csp_latency=1, misc=off, implementation=core}
      mask prompts: replication "replication factor"; csp_latency "latency"; misc "misc support"; implementation "delay implementation"
      mask help: Output bus formed by replicating input bus a number of times
      mask init:
      | bus_replicate_init(gcb, ...
      |     'replication', replication, ...
      |     'csp_latency', csp_latency, ...
      |     'implementation', implementation, ...
      |     'misc', misc);
      mask TypeOptions implementation: core | behavioral
  convert_im : xbsIndex_r4/Convert  gui_display_data_type=Fixed-point  arith_type="Signed  (2's comp)"  n_bits=18  bin_pt=17  float_type=Single  exp_bits=8  fraction_bits=24  quantization="Round  (unbiased: +/- Inf)"  overflow=Wrap  en=off  latency=7  pipeline=on  dbl_ovrd=off  block_type=convert
  convert_re : xbsIndex_r4/Convert  gui_display_data_type=Fixed-point  arith_type="Signed  (2's comp)"  n_bits=18  bin_pt=17  float_type=Single  exp_bits=8  fraction_bits=24  quantization="Round  (unbiased: +/- Inf)"  overflow=Wrap  en=off  latency=7  pipeline=on  dbl_ovrd=off  block_type=convert
  imim : xbsIndex_r4/Mult  precision=Full  arith_type="Signed  (2's comp)"  n_bits=16  bin_pt=14  quantization=Truncate  overflow=Wrap  en=off  latency=7  use_behavioral_HDL=off  opt=Speed  use_embedded=on  optimum_pipeline=off  pipeline=on  dbl_ovrd=off  use_rpm=on  placement_style=Triangular  block_type=mult
  imre : xbsIndex_r4/Mult  precision=Full  arith_type="Signed  (2's comp)"  n_bits=16  bin_pt=14  quantization=Truncate  overflow=Wrap  en=off  latency=7  use_behavioral_HDL=off  opt=Speed  use_embedded=on  optimum_pipeline=off  pipeline=on  dbl_ovrd=off  use_rpm=on  placement_style=Triangular  block_type=mult
  reim : xbsIndex_r4/Mult  precision=Full  arith_type="Signed  (2's comp)"  n_bits=16  bin_pt=14  quantization=Truncate  overflow=Wrap  en=off  latency=7  use_behavioral_HDL=off  opt=Speed  use_embedded=on  optimum_pipeline=off  pipeline=on  dbl_ovrd=off  use_rpm=on  placement_style=Triangular  block_type=mult
  rere : xbsIndex_r4/Mult  precision=Full  arith_type="Signed  (2's comp)"  n_bits=16  bin_pt=14  quantization=Truncate  overflow=Wrap  en=off  latency=7  use_behavioral_HDL=off  opt=Speed  use_embedded=on  optimum_pipeline=off  pipeline=on  dbl_ovrd=off  use_rpm=on  placement_style=Triangular  block_type=mult
  ri_to_c : Subsystem  mask(ri_to_c){}
      mask help:
      | Concatenates real and imaginary inputs into a complex output.
      | Useful for simplifying interconnects.
      | See also: Complex to Real-Imag (c_to_ri)
      mask Help: eval('xlWeb(''http://casper.berkeley.edu/wiki/Ri_to_c'')')
  ab : Outport
  wires:
  a/1 -> a_replicate/1(in)
  b/1 -> b_replicate/1(in)
  a_replicate/1(out) -> a_expand/1(bus_in)
  b_replicate/1(out) -> b_expand/1(bus_in)
  a_expand/1(msb_out4) -> rere/1
  b_expand/1(msb_out4) -> rere/2
  a_expand/2(out3) -> imim/1
  b_expand/2(out3) -> imim/2
  a_expand/4(lsb_out1) -> imre/1
  b_expand/3(out2) -> imre/2
  a_expand/3(out2) -> reim/1
  b_expand/4(lsb_out1) -> reim/2
  rere/1 -> addsub_re/1
  imim/1 -> addsub_re/2
  imre/1 -> addsub_im/1
  reim/1 -> addsub_im/2
  addsub_re/1 -> convert_re/1
  addsub_im/1 -> convert_im/1
  convert_re/1 -> ri_to_c/1(re)
  convert_im/1 -> ri_to_c/2(im)
  ri_to_c/1(c) -> ab/1
